simulink model "HRES_ORC_PEM"  (R2025b)
settings: Solver=ode23t  StartTime=0.0  StopTime=35000  MaxStep=1728  RelTol=1e-3
model workspace (MAT data in the model file):
  CND_L = 10
  CND_T0 = 333.15
  CND_d = 0.012
  CND_n = 20
  CND_p0 = 150000
  GAS_Tmax = 430
  GAS_dT = 20
  GAS_kb = 0.04
  GAS_ki = 0.002
  GAS_kp = 0.05
  GAS_min = 0.02
  GAS_total = 5
  GAS_u0 = 0.05
  HRS_L = 10
  HRS_LG = 1
  HRS_d = 0.012
  HRS_n = 6
  HRS_nG = 25
  HRS_p0 = 0.3
  HRS_x0 = 0.2
  NOZ_kb = 0.025
  NOZ_ki = 0.0005
  NOZ_kp = 0.02
  NOZ_min = 0.01
  NOZ_u0 = 0.1
  ORC_T3set = 400
  ORC_Taux = -2
  ORC_Taux0 = 0
  ORC_kb = 0.4
  ORC_ki = 2e-07
  ORC_kp = 5e-07
  ORC_mdot0 = 0.2
  ORC_mmax = 1
  ORC_mmin = 0.01
  ORC_pset_MPa = 1
  RCV_V = 0.2
  RCV_frac0 = 0.5
  RCV_p0 = 0.15
  RCV_tau = 0.1
  TRB_Tref = 400
  TRB_mdot = 0.6
  TRB_pr = 6
values from neighbouring files (symbols this model uses):
  R_h2 = 4.12    [run_simulation.m]
libraries: fl_lib x62, nesl_utility x56, SimscapeFluids_lib x9, slpidlib x4, ee_lib x2
(part 5 of 5)

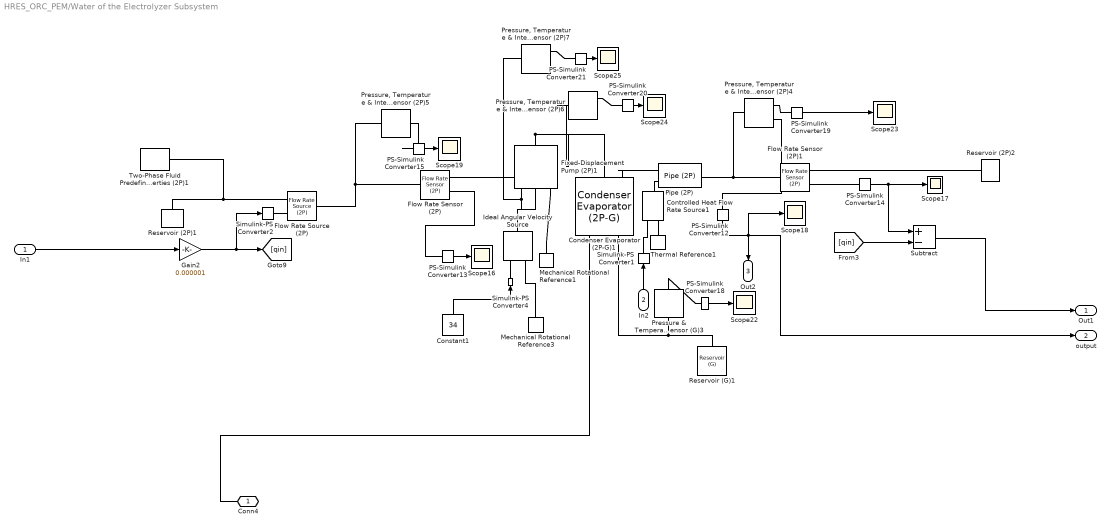
== system HRES_ORC_PEM/Water of the Electrolyzer Subsystem ==
  In1 : Inport
  In2 : Inport  Port=2
  Condenser Evaporator (2P-G)1 : SimscapeFluids_lib/Heat Exchangers/Two-Phase Fluid - Gas/Condenser Evaporator (2P-G)  flow_arrangement=fluids.heat_exchangers.enum.FlowArrangement2PG.Cross  cross_flow_arrangement=fluids.heat_exchangers.enum.CrossFlowArrangement2PG.UnmixedUnmixed  R_wall=0 K/kW  wall_thermal_mass=false  mass_wall=1 kg  cp_wall=490 J/(K*kg)  area_A1=0.01 m^2  area_B1=0.01 m^2  area_A2=0.01 m^2  area_B2=0.01 m^2  tube_num_2P=20  tube_length_2P=1 m  tube_cross_section_2P=fluids.heat_exchangers.enum.TubeCrossSection.Circular  tube_diameter_2P=0.1 m  tube_width_2P=0.05 m  tube_height_2P=0.05 m  tube_inner_diameter_2P=0.05 m  tube_outer_diameter_2P=0.1 m  tube_flow_area_2P=0.002 m^2  tube_wetted_perimeter_2P=0.15 m  tube_heat_perimeter_2P=0.15 m  tube_pressure_loss_spec_2P=fluids.heat_exchangers.enum.TubePressureLossSpec2P.Haaland  tube_loss_coeff_2P=10  tube_local_pressure_loss_spec_2P=fluids.heat_exchangers.enum.LocalLossSpec.AggregateLength  tube_length_add_2P=0.1 m  tube_local_loss_coefficient_2P=0.1  tube_roughness_pressure_2P=15e-6 m  tube_Re_lam_pressure_2P=2000  tube_Re_tur_pressure_2P=4000  tube_shape_factor_generic_2P=64  tube_heat_coeff_spec_2P=fluids.heat_exchangers.enum.TubeHeatCoeffSpec2P.GneilinskiCavalliniZecchin  tube_colburn_coeff_liq_2P=[.023, .8, .33]  tube_colburn_coeff_mix_2P=[.05, .8, .33]  tube_colburn_coeff_vap_2P=[.023, .8, .33]  tube_roughness_heat_2P=15e-6 m  tube_Re_lam_heat_2P=2000  tube_Re_tur_heat_2P=4000  tube_Nu_lam_generic_2P=3.66  fouling_factor_2P=0.1 K*m^2/kW  fin_area_2P=0 m^2  fin_efficiency_2P=0.5  energy_spec_2P=foundation.enum.energy_spec.temperature  p_init_2P=0.6 MPa  T_init_2P=293.15 K  x_init_2P=0.5  alpha_init_2P=0.5  h_init_2P=1500 kJ/kg  u_init_2P=1500 kJ/kg  flow_geometry_G=fluids.heat_exchangers.enum.FlowGeometryG.InsideTubes  tube_num_G=20  tube_length_G=1 m  tube_cross_section_G=fluids.heat_exchangers.enum.TubeCrossSection.Circular  tube_diameter_G=0.05 m  tube_width_G=0.05 m  tube_height_G=0.05 m  tube_inner_diameter_G=0.05 m  tube_outer_diameter_G=0.1 m  tube_flow_area_G=0.002 m^2  tube_wetted_perimeter_G=0.15 m  tube_heat_perimeter_G=0.15 m  tube_pressure_loss_spec_G=fluids.heat_exchangers.enum.TubePressureLossSpec.Haaland  tube_loss_coeff_G=10  tube_local_pressure_loss_spec_G=fluids.heat_exchangers.enum.LocalLossSpec.AggregateLength  tube_length_add_G=0.1 m  tube_local_loss_coefficient_G=0.1  tube_roughness_pressure_G=15e-6 m  tube_Re_lam_pressure_G=2000  tube_Re_tur_pressure_G=4000  tube_shape_factor_generic_G=64  tube_heat_coeff_spec_G=fluids.heat_exchangers.enum.TubeHeatCoeffSpec.Gneilinski  tube_colburn_coeff_G=[.023, .8, .33]  tube_roughness_heat_G=15e-6 m  tube_Re_lam_heat_G=2000  tube_Re_tur_heat_G=4000  tube_Nu_lam_generic_G=3.66  bank_arrangement_G=fluids.heat_exchangers.enum.BankArrangement.Inline  bank_num_rows_G=5  bank_tubes_per_row_G=5  bank_width_G=1 m  bank_tube_diameter_G=0.05 m  bank_longitudinal_pitch_G=0.15 m  bank_transverse_pitch_G=0.15 m  bank_pressure_loss_spec_G=fluids.heat_exchangers.enum.BankPressureLossSpec.Martin  bank_euler_G=10  bank_heat_coeff_spec_G=fluids.heat_exchangers.enum.BankHeatCoeffSpec.Martin  bank_colburn_coeff_G=[.27, .63, .36]  generic_flow_area_G=0.01 m^2  generic_heat_area_G=2 m^2  generic_volume_G=0.05 m^3  generic_loss_coeff_G=10  generic_colburn_coeff_G=[.023, .8, .33]  fouling_factor_G=0.1 K*m^2/kW  fin_area_G=0 m^2  fin_efficiency_G=0.5  p_init_G=0.101325 MPa  T_init_G=250 K
      settings: InternalSimscapePortConfiguration="{\"Bottom\":[],\"Left\":[{\"id\":\"A1\",\"label\":\"A1\",\"type\":\"foundation.two_phase_fluid.two_phase_fluid\"},{\"id\":\"B1\",\"label\":\"B1\",\"type\":\"foundation.two_phase_fluid.two_phase_fluid\"}],\"Right\":[{\"id\":\"A2\",\"label\":\"A2\",\"type\":\"foundation.gas.gas\"},{\"id\":\"B2\",\"label\":\"B2\",\"type\":\"foundation.gas.gas\"}],\"Top\":[{\"id\":\"Z\",\"label\":\"Z\",\"type\":\"output\"}]}"
  Constant1 : Constant  Value=34
  Controlled Heat Flow Rate Source1 : fl_lib/Thermal/Thermal Sources/Controlled Heat Flow Rate Source
  Fixed-Displacement Pump (2P)1 : SimscapeFluids_lib/Two-Phase Fluid/Fluid Machines/Fixed-Displacement Pump (2P)  leakage_friction_spec=fluids.two_phase_fluid.fluid_machines.enum.PumpMotorLossSpec.Analytical  displacement=20 cm^3/rev  omega_nominal=10 rad/s  p_nominal=0.3 MPa  mu_nominal=0.9 cP  vol_eff_nominal=0.85  mech_eff_nominal=0.80  no_load_torque=0 N*m  p_diff_eff_TLU=[.1, 1, 2] MPa  omega_eff_TLU=[250, 500, 1000, 2000, 3000, 4000] rpm  vol_eff_TLU=[.816, .908, .954, .977, .981, .984; .325, .663, .831, .916, .925, .946; .137, .568, .78, .892, .893, .91]  mech_eff_TLU=[.996, .996, .996, .996, .996, .996; .988, .989, .989, .989, .989, .99; .981, .981, .982, .982, .983, .984]  p_diff_loss_TLU=[.1, 1, 2] MPa  omega_loss_TLU=[250, 500, 1000, 2000, 3000, 4000] rpm  vol_loss_TLU=1e-3 * [.023, .023, .023, .023, .0285, .032; .0844, .0842, .0845, .084, .1125, .108; .1079, .108, .11, .108, .1605, .18] m^3/s  mech_loss_TLU=[.002, .002, .002, .002, .002, .002; .0607, .0556, .0556, .0556, .0556, .0505; .1937, .1937, .1833, .1833, .1729, .1626] N*m  vol_eff_min=1e-3  vol_eff_max=1  mech_eff_min=1e-3  mech_eff_max=1  pressure_threshold=1e-3 MPa  omega_threshold=100 rpm  area=0.001 m^2  liquid_check=simscape.enum.assert.action.warn  supplied_range_check=simscape.enum.assert.action.none  pump_mode_check=simscape.enum.assert.action.none
      settings: LogSimulationData=on  InternalSimscapePortConfiguration="{\"Bottom\":[{\"id\":\"A\",\"label\":\"A\",\"type\":\"foundation.two_phase_fluid.two_phase_fluid\"}],\"Left\":[],\"Right\":[{\"id\":\"R\",\"label\":\"R\",\"type\":\"foundation.mechanical.rotational.rotational\"},{\"id\":\"C\",\"label\":\"C\",\"type\":\"foundation.mechanical.rotational.rotational\"}],\"Top\":[{\"id\":\"B\",\"label\":\"B\",\"type\":\"foundation.two_phase_fluid.two_phase_fluid\"}]}"
  Flow Rate Sensor (2P) : fl_lib/Two-Phase Fluid/Sensors/Flow Rate Sensor (2P)  mass_flow_measure=true  volumetric_flow_measure=false  energy_flow_measure=false
      settings: InternalSimscapePortConfiguration="{\"Bottom\":[],\"Left\":[{\"id\":\"A\",\"label\":\"A\",\"type\":\"foundation.two_phase_fluid.two_phase_fluid\"}],\"Right\":[{\"id\":\"B\",\"label\":\"B\",\"type\":\"foundation.two_phase_fluid.two_phase_fluid\"},{\"id\":\"M\",\"label\":\"M\",\"type\":\"output\"}],\"Top\":[]}"
  Flow Rate Sensor (2P)1 : fl_lib/Two-Phase Fluid/Sensors/Flow Rate Sensor (2P)  mass_flow_measure=false  volumetric_flow_measure=true  energy_flow_measure=false
      settings: InternalSimscapePortConfiguration="{\"Bottom\":[],\"Left\":[{\"id\":\"A\",\"label\":\"A\",\"type\":\"foundation.two_phase_fluid.two_phase_fluid\"}],\"Right\":[{\"id\":\"B\",\"label\":\"B\",\"type\":\"foundation.two_phase_fluid.two_phase_fluid\"},{\"id\":\"V\",\"label\":\"V\",\"type\":\"output\"}],\"Top\":[]}"
  Flow Rate Source (2P) : fl_lib/Two-Phase Fluid/Sources/Flow Rate Source (2P)  source_type=foundation.enum.constant_controlled.controlled  flow_type=foundation.enum.mass_volumetric_flow.mass  mass_flow=0 kg/s  volumetric_flow=0 m^3/s  power_spec=foundation.enum.power_spec.isentropic  area_A=0.01 m^2  area_B=0.01 m^2
      settings: InternalSimscapePortConfiguration="{\"Bottom\":[],\"Left\":[{\"id\":\"A\",\"label\":\"A\",\"type\":\"foundation.two_phase_fluid.two_phase_fluid\"},{\"id\":\"M\",\"label\":\"M\",\"type\":\"input\"}],\"Right\":[{\"id\":\"B\",\"label\":\"B\",\"type\":\"foundation.two_phase_fluid.two_phase_fluid\"}],\"Top\":[]}"
  Gain2 : Gain  Gain=0.000001
  Ideal Angular Velocity Source : fl_lib/Mechanical/Mechanical Sources/Ideal Angular Velocity Source
  Mechanical Rotational Reference1 : fl_lib/Mechanical/Rotational Elements/Mechanical Rotational Reference
  Mechanical Rotational Reference3 : fl_lib/Mechanical/Rotational Elements/Mechanical Rotational Reference
  PS-Simulink Converter12 : nesl_utility/PS-Simulink Converter  PhysicalDomain=network_engine_domain  SubClassName=ps_output  LeftPortType=input  RightPortType=output  PseudoPeriodic=off  Frequencies=[]  VectorFormat=inherit  Unit=K  AffineConversion=off
  PS-Simulink Converter13 : nesl_utility/PS-Simulink Converter  PhysicalDomain=network_engine_domain  SubClassName=ps_output  LeftPortType=input  RightPortType=output  PseudoPeriodic=off  Frequencies=[]  VectorFormat=inherit  Unit=inherit  AffineConversion=off
  PS-Simulink Converter14 : nesl_utility/PS-Simulink Converter  PhysicalDomain=network_engine_domain  SubClassName=ps_output  LeftPortType=input  RightPortType=output  PseudoPeriodic=off  Frequencies=[]  VectorFormat=inherit  Unit=m^3/s  AffineConversion=off
  PS-Simulink Converter15 : nesl_utility/PS-Simulink Converter  PhysicalDomain=network_engine_domain  SubClassName=ps_output  LeftPortType=input  RightPortType=output  PseudoPeriodic=off  Frequencies=[]  VectorFormat=inherit  Unit=inherit  AffineConversion=off
  PS-Simulink Converter18 : nesl_utility/PS-Simulink Converter  PhysicalDomain=network_engine_domain  SubClassName=ps_output  LeftPortType=input  RightPortType=output  PseudoPeriodic=off  Frequencies=[]  VectorFormat=inherit  Unit=K  AffineConversion=off
  PS-Simulink Converter19 : nesl_utility/PS-Simulink Converter  PhysicalDomain=network_engine_domain  SubClassName=ps_output  LeftPortType=input  RightPortType=output  PseudoPeriodic=off  Frequencies=[]  VectorFormat=inherit  Unit=inherit  AffineConversion=off
  PS-Simulink Converter20 : nesl_utility/PS-Simulink Converter  PhysicalDomain=network_engine_domain  SubClassName=ps_output  LeftPortType=input  RightPortType=output  PseudoPeriodic=off  Frequencies=[]  VectorFormat=inherit  Unit=Pa  AffineConversion=off
  PS-Simulink Converter21 : nesl_utility/PS-Simulink Converter  PhysicalDomain=network_engine_domain  SubClassName=ps_output  LeftPortType=input  RightPortType=output  PseudoPeriodic=off  Frequencies=[]  VectorFormat=inherit  Unit=Pa  AffineConversion=off
  Pipe (2P) : fl_lib/Two-Phase Fluid/Elements/Pipe (2P)  length=5 m  area=0.01 m^2  Dh=0.1 m  length_add=0.1 m  roughness=15e-6 m  Re_lam=2000  Re_tur=4000  shape_factor=64  Nu_lam=3.66  inertia=false  energy_spec=foundation.enum.energy_spec.temperature  p_init=0.101325 MPa  T_init=293.15 K  x_init=0.5  alpha_init=0.5  h_init=1500 kJ/kg  u_init=1500 kJ/kg  mdot_init=0 kg/s  time_constant=0.1 s
      settings: InternalSimscapePortConfiguration="{\"Bottom\":[],\"Left\":[{\"id\":\"A\",\"label\":\"A\",\"type\":\"foundation.two_phase_fluid.two_phase_fluid\"},{\"id\":\"H\",\"label\":\"H\",\"type\":\"foundation.thermal.thermal\"}],\"Right\":[{\"id\":\"B\",\"label\":\"B\",\"type\":\"foundation.two_phase_fluid.two_phase_fluid\"}],\"Top\":[]}"
  Pressure & Temperature Sensor (G)3 : fl_lib/Gas/Sensors/Pressure & Temperature Sensor (G)  reference=foundation.enum.MeasurementReference.absolute  pressure=false  pressure_spec=foundation.enum.PressureMeasementSpec.Absolute  temperature=true
      settings: InternalSimscapePortConfiguration="{\"Bottom\":[{\"id\":\"T\",\"label\":\"T\",\"type\":\"output\"}],\"Left\":[{\"id\":\"A\",\"label\":\"A\",\"type\":\"foundation.gas.gas\"}],\"Right\":[],\"Top\":[]}"
  "Pressure, Temperature & Internal Energy Sensor (2P)4" : fl_lib/Two-Phase Fluid/Sensors/Pressure, Temperature & Internal Energy Sensor (2P)  reference=foundation.enum.MeasurementReference.absolute  pressure=true  pressure_spec=foundation.enum.PressureMeasementSpec.Absolute  temperature=true  internal_energy=false
      settings: InternalSimscapePortConfiguration="{\"Bottom\":[{\"id\":\"T\",\"label\":\"T\",\"type\":\"output\"}],\"Left\":[{\"id\":\"A\",\"label\":\"A\",\"type\":\"foundation.two_phase_fluid.two_phase_fluid\"}],\"Right\":[{\"id\":\"Pa\",\"label\":\"Pa\",\"type\":\"output\"}],\"Top\":[]}"
  "Pressure, Temperature & Internal Energy Sensor (2P)5" : fl_lib/Two-Phase Fluid/Sensors/Pressure, Temperature & Internal Energy Sensor (2P)  reference=foundation.enum.MeasurementReference.absolute  pressure=false  pressure_spec=foundation.enum.PressureMeasementSpec.Absolute  temperature=true  internal_energy=false
      settings: InternalSimscapePortConfiguration="{\"Bottom\":[{\"id\":\"T\",\"label\":\"T\",\"type\":\"output\"}],\"Left\":[{\"id\":\"A\",\"label\":\"A\",\"type\":\"foundation.two_phase_fluid.two_phase_fluid\"}],\"Right\":[],\"Top\":[]}"
  "Pressure, Temperature & Internal Energy Sensor (2P)6" : fl_lib/Two-Phase Fluid/Sensors/Pressure, Temperature & Internal Energy Sensor (2P)  reference=foundation.enum.MeasurementReference.absolute  pressure=true  pressure_spec=foundation.enum.PressureMeasementSpec.Absolute  temperature=true  internal_energy=false
      settings: InternalSimscapePortConfiguration="{\"Bottom\":[{\"id\":\"T\",\"label\":\"T\",\"type\":\"output\"}],\"Left\":[{\"id\":\"A\",\"label\":\"A\",\"type\":\"foundation.two_phase_fluid.two_phase_fluid\"}],\"Right\":[{\"id\":\"Pa\",\"label\":\"Pa\",\"type\":\"output\"}],\"Top\":[]}"
  "Pressure, Temperature & Internal Energy Sensor (2P)7" : fl_lib/Two-Phase Fluid/Sensors/Pressure, Temperature & Internal Energy Sensor (2P)  reference=foundation.enum.MeasurementReference.absolute  pressure=true  pressure_spec=foundation.enum.PressureMeasementSpec.Absolute  temperature=true  internal_energy=false
      settings: InternalSimscapePortConfiguration="{\"Bottom\":[{\"id\":\"T\",\"label\":\"T\",\"type\":\"output\"}],\"Left\":[{\"id\":\"A\",\"label\":\"A\",\"type\":\"foundation.two_phase_fluid.two_phase_fluid\"}],\"Right\":[{\"id\":\"Pa\",\"label\":\"Pa\",\"type\":\"output\"}],\"Top\":[]}"
  Reservoir (2P)1 : fl_lib/Two-Phase Fluid/Elements/Reservoir (2P)  pressure_spec=foundation.enum.ReservoirPressureSpec2P.Specified  reservoir_pressure=1 bar  reservoir_condensing_temperature=373.15 K  reservoir_evaporating_temperature=373.15 K  energy_spec=foundation.enum.ReservoirEnergySpec2P.Temperature  reservoir_temperature=300 K  reservoir_quality=0.5  reservoir_void_fraction=0.5  reservoir_enthalpy=1500 kJ/kg  reservoir_internal_energy=1500 kJ/kg  reservoir_subcooling=5 deltaK  reservoir_superheating=5 deltaK  area_A=0.01 m^2
  Reservoir (2P)2 : fl_lib/Two-Phase Fluid/Elements/Reservoir (2P)  pressure_spec=foundation.enum.ReservoirPressureSpec2P.Specified  reservoir_pressure=5 bar  reservoir_condensing_temperature=373.15 K  reservoir_evaporating_temperature=373.15 K  energy_spec=foundation.enum.ReservoirEnergySpec2P.Temperature  reservoir_temperature=370 K  reservoir_quality=0.5  reservoir_void_fraction=0.5  reservoir_enthalpy=1500 kJ/kg  reservoir_internal_energy=1500 kJ/kg  reservoir_subcooling=5 deltaK  reservoir_superheating=5 deltaK  area_A=0.01 m^2
  Reservoir (G)1 : fl_lib/Gas/Elements/Reservoir (G)  pressure_spec=foundation.enum.pressure_spec.atmospheric  reservoir_pressure=0.101325 MPa  reservoir_temperature=293.15 K  area_A=0.01 m^2
  Scope{16..19,22..25} (8 alike) : Scope
      Scope16 settings: ActiveDisplayYMinimum=-4.6224964079817441E-7  ActiveDisplayYMaximum=4.160246767183571E-6  DataLoggingVariableName=ScopeData18
      Scope17 settings: ActiveDisplayYMinimum=-0.00043435582595641739  ActiveDisplayYMaximum=0.0035069615419707017  DataLoggingVariableName=ScopeData19
      Scope18 settings: ActiveDisplayYMinimum=296.23361130845234  ActiveDisplayYMaximum=380.90999792555522  DataLoggingVariableName=ScopeData15
      Scope19 settings: ActiveDisplayYMinimum=269.69619495924803  ActiveDisplayYMaximum=487.04134680243965  DataLoggingVariableName=ScopeData17
      Scope22 settings: ActiveDisplayYMinimum=-544.89033893414171  ActiveDisplayYMaximum=1096.9615501303642  DataLoggingVariableName=ScopeData22
      Scope23 settings: ActiveDisplayYMinimum=0.099971820776618758  ActiveDisplayYMaximum=0.10001711054963275  DataLoggingVariableName=ScopeData23
      Scope24 settings: ActiveDisplayYMinimum=499999.999811996  ActiveDisplayYMaximum=500000.00715155876  DataLoggingVariableName=ScopeData24
      Scope25 settings: ActiveDisplayYMinimum=499999.999811996  ActiveDisplayYMaximum=500000.00715155876  DataLoggingVariableName=ScopeData25
  Simulink-PS Converter1 : nesl_utility/Simulink-PS Converter  PhysicalDomain=network_engine_domain  SubClassName=ps_input  LeftPortType=input  RightPortType=output  PseudoPeriodic=off  Frequencies=[]  NoiseDistribution=none  NoiseParameters=[]  Unit=W  AffineConversion=off  FilteringAndDerivatives=provide  SimscapeFilterOrder=1  InputFilterTimeConstant=0.001  UdotUserProvided=0
  Simulink-PS Converter2 : nesl_utility/Simulink-PS Converter  PhysicalDomain=network_engine_domain  SubClassName=ps_input  LeftPortType=input  RightPortType=output  PseudoPeriodic=off  Frequencies=[]  NoiseDistribution=none  NoiseParameters=[]  Unit=1  AffineConversion=off  FilteringAndDerivatives=provide  SimscapeFilterOrder=1  InputFilterTimeConstant=0.001  UdotUserProvided=0
  Simulink-PS Converter4 : nesl_utility/Simulink-PS Converter  PhysicalDomain=network_engine_domain  SubClassName=ps_input  LeftPortType=input  RightPortType=output  PseudoPeriodic=off  Frequencies=[]  NoiseDistribution=none  NoiseParameters=[]  Unit=1  AffineConversion=off  FilteringAndDerivatives=provide  SimscapeFilterOrder=1  InputFilterTimeConstant=0.001  UdotUserProvided=0
  Subtract : Sum  Inputs=+-
  Thermal Reference1 : fl_lib/Thermal/Thermal Elements/Thermal Reference
  Two-Phase Fluid Predefined Properties (2P)1 : SimscapeFluids_lib/Two-Phase Fluid/Utilities/Two-Phase Fluid Predefined Properties (2P)  fluid=fluids.two_phase_fluid.utilities.enum.Fluid.Water  p_atm=0.101325 MPa  properties_range_check=simscape.enum.assert.action.error  q_rev=0.01 Pa
  Conn4 : PMIOPort  Side=Right
  Out1 : Outport
  output : Outport  Port=2
  Out2 : Outport  Port=3
  wires:
  PS-Simulink Converter13/1 -> Scope16/1
  PS-Simulink Converter15/1 -> Scope19/1
  PS-Simulink Converter21/1 -> Scope25/1
  PS-Simulink Converter19/1 -> Scope23/1
  PS-Simulink Converter12/1 -> output/1, Scope18/1, Out2/1
  PS-Simulink Converter20/1 -> Scope24/1
  Constant1/1 -> Simulink-PS Converter4/1
  PS-Simulink Converter14/1 -> Subtract/1, Scope17/1
  PS-Simulink Converter18/1 -> Scope22/1
  [qin] -> Subtract/2
  In1/1 -> Gain2/1
  Gain2/1 -> Simulink-PS Converter2/1, [qin]
  Subtract/1 -> Out1/1
  In2/1 -> Simulink-PS Converter1/1
  connections:
  PS-Simulink Converter12/LConn1 -- "Pressure, Temperature & Internal Energy Sensor (2P)4"/RConn2
  "Pressure, Temperature & Internal Energy Sensor (2P)5"/LConn1 -- Flow Rate Sensor (2P)/LConn1 -- Flow Rate Source (2P)/RConn1
  Reservoir (G)1/LConn1 -- Pressure & Temperature Sensor (G)3/LConn1 -- Condenser Evaporator (2P-G)1/RConn1
  Mechanical Rotational Reference3/LConn1 -- Ideal Angular Velocity Source/RConn2
  Ideal Angular Velocity Source/RConn1 -- Simulink-PS Converter4/RConn1
  Two-Phase Fluid Predefined Properties (2P)1/RConn1 -- Reservoir (2P)1/LConn1 -- Flow Rate Source (2P)/LConn1
  PS-Simulink Converter21/LConn1 -- "Pressure, Temperature & Internal Energy Sensor (2P)7"/RConn1
  Mechanical Rotational Reference1/LConn1 -- Fixed-Displacement Pump (2P)1/RConn1
  PS-Simulink Converter20/LConn1 -- "Pressure, Temperature & Internal Energy Sensor (2P)6"/RConn1
  Flow Rate Sensor (2P)/RConn2 -- PS-Simulink Converter13/LConn1
  PS-Simulink Converter15/LConn1 -- "Pressure, Temperature & Internal Energy Sensor (2P)5"/RConn1
  Flow Rate Source (2P)/LConn2 -- Simulink-PS Converter2/RConn1
  PS-Simulink Converter19/LConn1 -- "Pressure, Temperature & Internal Energy Sensor (2P)4"/RConn1
  "Pressure, Temperature & Internal Energy Sensor (2P)4"/LConn1 -- Flow Rate Sensor (2P)1/LConn1 -- Pipe (2P)/RConn1
  Pipe (2P)/LConn1 -- Condenser Evaporator (2P-G)1/LConn1
  Pressure & Temperature Sensor (G)3/RConn1 -- PS-Simulink Converter18/LConn1
  Fixed-Displacement Pump (2P)1/RConn3 -- Flow Rate Sensor (2P)/RConn1 -- "Pressure, Temperature & Internal Energy Sensor (2P)7"/LConn1
  PS-Simulink Converter14/LConn1 -- Flow Rate Sensor (2P)1/RConn2
  Fixed-Displacement Pump (2P)1/LConn1 -- "Pressure, Temperature & Internal Energy Sensor (2P)6"/LConn1 -- Condenser Evaporator (2P-G)1/LConn2
  Conn4/RConn1 -- Condenser Evaporator (2P-G)1/RConn2
  Flow Rate Sensor (2P)1/RConn1 -- Reservoir (2P)2/LConn1
  Fixed-Displacement Pump (2P)1/RConn2 -- Ideal Angular Velocity Source/LConn1
  Thermal Reference1/LConn1 -- Controlled Heat Flow Rate Source1/RConn2
  Simulink-PS Converter1/RConn1 -- Controlled Heat Flow Rate Source1/RConn1
  Controlled Heat Flow Rate Source1/LConn1 -- Pipe (2P)/LConn2

== system HRES_ORC_PEM/ORC/Load Torque ==
  In1 : Inport
  In2 : Inport  Port=2
  In3 : Inport  Port=3
  Switch : Switch  Threshold=1000  SaturateOnIntegerOverflow=off  InputSameDT=off
  Out1 : Outport
  wires:
  In1/1 -> Switch/3
  Switch/1 -> Out1/1
  In2/1 -> Switch/2
  In3/1 -> Switch/1

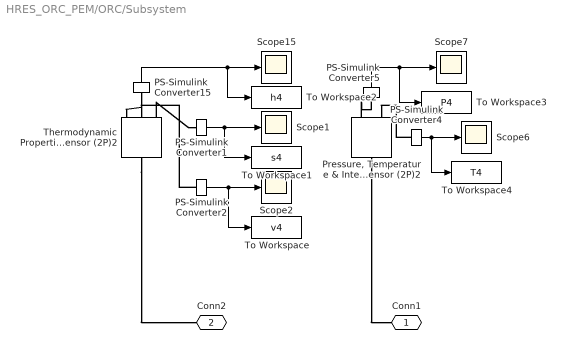
== system HRES_ORC_PEM/ORC/Subsystem ==
  PS-Simulink Converter1 : nesl_utility/PS-Simulink Converter  PhysicalDomain=network_engine_domain  SubClassName=ps_output  LeftPortType=input  RightPortType=output  PseudoPeriodic=off  Frequencies=[]  VectorFormat=inherit  Unit=J/(kg*K)  AffineConversion=off
  PS-Simulink Converter15 : nesl_utility/PS-Simulink Converter  PhysicalDomain=network_engine_domain  SubClassName=ps_output  LeftPortType=input  RightPortType=output  PseudoPeriodic=off  Frequencies=[]  VectorFormat=inherit  Unit=kJ/kg  AffineConversion=off
  PS-Simulink Converter2 : nesl_utility/PS-Simulink Converter  PhysicalDomain=network_engine_domain  SubClassName=ps_output  LeftPortType=input  RightPortType=output  PseudoPeriodic=off  Frequencies=[]  VectorFormat=inherit  Unit=m^3/kg  AffineConversion=off
  PS-Simulink Converter4 : nesl_utility/PS-Simulink Converter  PhysicalDomain=network_engine_domain  SubClassName=ps_output  LeftPortType=input  RightPortType=output  PseudoPeriodic=off  Frequencies=[]  VectorFormat=inherit  Unit=K  AffineConversion=off
  PS-Simulink Converter5 : nesl_utility/PS-Simulink Converter  PhysicalDomain=network_engine_domain  SubClassName=ps_output  LeftPortType=input  RightPortType=output  PseudoPeriodic=off  Frequencies=[]  VectorFormat=inherit  Unit=Pa  AffineConversion=off
  "Pressure, Temperature & Internal Energy Sensor (2P)2" : fl_lib/Two-Phase Fluid/Sensors/Pressure, Temperature & Internal Energy Sensor (2P)  reference=foundation.enum.MeasurementReference.absolute  pressure=true  pressure_spec=foundation.enum.PressureMeasementSpec.Absolute  temperature=true  internal_energy=false
      settings: InternalSimscapePortConfiguration="{\"Bottom\":[{\"id\":\"T\",\"label\":\"T\",\"type\":\"output\"}],\"Left\":[{\"id\":\"A\",\"label\":\"A\",\"type\":\"foundation.two_phase_fluid.two_phase_fluid\"}],\"Right\":[{\"id\":\"Pa\",\"label\":\"Pa\",\"type\":\"output\"}],\"Top\":[]}"
  Scope{1..2,6..7,15} (5 alike) : Scope
      Scope1 settings: ActiveDisplayYMinimum=375.93552600794726  ActiveDisplayYMaximum=401.12975249571122  DataLoggingVariableName=ScopeData27
      Scope15 settings: ActiveDisplayYMinimum=260.896690836373  ActiveDisplayYMaximum=388.3546236466708  DataLoggingVariableName=ScopeData20
      Scope2 settings: ActiveDisplayYMinimum=375.93552600794726  ActiveDisplayYMaximum=401.12975249571122  DataLoggingVariableName=ScopeData28
      Scope6 settings: ActiveDisplayYMinimum=-1  ActiveDisplayYMaximum=1  DataLoggingVariableName=ScopeData6
      Scope7 settings: ActiveDisplayYMinimum=287076.80367816926  ActiveDisplayYMaximum=1.2873113409355804E+6  DataLoggingVariableName=ScopeData7
  Thermodynamic Properties Sensor (2P)2 : fl_lib/Two-Phase Fluid/Sensors/Thermodynamic Properties Sensor (2P)  temperature=false  enthalpy=true  density=false  specific_volume=true  entropy=true
      settings: InternalSimscapePortConfiguration="{\"Bottom\":[{\"id\":\"V\",\"label\":\"v\",\"type\":\"output\"},{\"id\":\"S\",\"label\":\"s\",\"type\":\"output\"}],\"Left\":[{\"id\":\"A\",\"label\":\"A\",\"type\":\"foundation.two_phase_fluid.two_phase_fluid\"}],\"Right\":[{\"id\":\"H\",\"label\":\"h\",\"type\":\"output\"}],\"Top\":[]}"
  To Workspace : ToWorkspace  VariableName=v4  SampleTime=-1
  To Workspace1 : ToWorkspace  VariableName=s4  SampleTime=-1
  To Workspace2 : ToWorkspace  VariableName=h4  SampleTime=-1
  To Workspace3 : ToWorkspace  VariableName=P4  SampleTime=-1
  To Workspace4 : ToWorkspace  VariableName=T4  SampleTime=-1
  Conn1 : PMIOPort  Side=Left
  Conn2 : PMIOPort  Port=2  Side=Left
  wires:
  PS-Simulink Converter15/1 -> To Workspace2/1, Scope15/1
  PS-Simulink Converter5/1 -> To Workspace3/1, Scope7/1
  PS-Simulink Converter1/1 -> To Workspace1/1, Scope1/1
  PS-Simulink Converter2/1 -> To Workspace/1, Scope2/1
  PS-Simulink Converter4/1 -> To Workspace4/1, Scope6/1
  connections:
  PS-Simulink Converter4/LConn1 -- "Pressure, Temperature & Internal Energy Sensor (2P)2"/RConn2
  PS-Simulink Converter15/LConn1 -- Thermodynamic Properties Sensor (2P)2/RConn1
  Thermodynamic Properties Sensor (2P)2/LConn1 -- Conn2/RConn1
  "Pressure, Temperature & Internal Energy Sensor (2P)2"/RConn1 -- PS-Simulink Converter5/LConn1
  "Pressure, Temperature & Internal Energy Sensor (2P)2"/LConn1 -- Conn1/RConn1
  Thermodynamic Properties Sensor (2P)2/RConn3 -- PS-Simulink Converter1/LConn1
  PS-Simulink Converter2/LConn1 -- Thermodynamic Properties Sensor (2P)2/RConn2

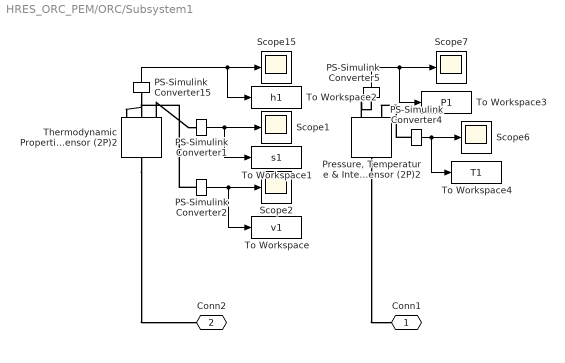
== system HRES_ORC_PEM/ORC/Subsystem1 ==
  PS-Simulink Converter1 : nesl_utility/PS-Simulink Converter  PhysicalDomain=network_engine_domain  SubClassName=ps_output  LeftPortType=input  RightPortType=output  PseudoPeriodic=off  Frequencies=[]  VectorFormat=inherit  Unit=J/(kg*K)  AffineConversion=off
  PS-Simulink Converter15 : nesl_utility/PS-Simulink Converter  PhysicalDomain=network_engine_domain  SubClassName=ps_output  LeftPortType=input  RightPortType=output  PseudoPeriodic=off  Frequencies=[]  VectorFormat=inherit  Unit=kJ/kg  AffineConversion=off
  PS-Simulink Converter2 : nesl_utility/PS-Simulink Converter  PhysicalDomain=network_engine_domain  SubClassName=ps_output  LeftPortType=input  RightPortType=output  PseudoPeriodic=off  Frequencies=[]  VectorFormat=inherit  Unit=m^3/kg  AffineConversion=off
  PS-Simulink Converter4 : nesl_utility/PS-Simulink Converter  PhysicalDomain=network_engine_domain  SubClassName=ps_output  LeftPortType=input  RightPortType=output  PseudoPeriodic=off  Frequencies=[]  VectorFormat=inherit  Unit=K  AffineConversion=off
  PS-Simulink Converter5 : nesl_utility/PS-Simulink Converter  PhysicalDomain=network_engine_domain  SubClassName=ps_output  LeftPortType=input  RightPortType=output  PseudoPeriodic=off  Frequencies=[]  VectorFormat=inherit  Unit=Pa  AffineConversion=off
  "Pressure, Temperature & Internal Energy Sensor (2P)2" : fl_lib/Two-Phase Fluid/Sensors/Pressure, Temperature & Internal Energy Sensor (2P)  reference=foundation.enum.MeasurementReference.absolute  pressure=true  pressure_spec=foundation.enum.PressureMeasementSpec.Absolute  temperature=true  internal_energy=false
      settings: InternalSimscapePortConfiguration="{\"Bottom\":[{\"id\":\"T\",\"label\":\"T\",\"type\":\"output\"}],\"Left\":[{\"id\":\"A\",\"label\":\"A\",\"type\":\"foundation.two_phase_fluid.two_phase_fluid\"}],\"Right\":[{\"id\":\"Pa\",\"label\":\"Pa\",\"type\":\"output\"}],\"Top\":[]}"
  Scope{1..2,6..7,15} (5 alike) : Scope
      Scope1 settings: ActiveDisplayYMinimum=375.93552600794726  ActiveDisplayYMaximum=401.12975249571122  DataLoggingVariableName=ScopeData27
      Scope15 settings: ActiveDisplayYMinimum=375.93552600794726  ActiveDisplayYMaximum=401.12975249571122  DataLoggingVariableName=ScopeData20
      Scope2 settings: ActiveDisplayYMinimum=375.93552600794726  ActiveDisplayYMaximum=401.12975249571122  DataLoggingVariableName=ScopeData28
      Scope6 settings: ActiveDisplayYMinimum=326.971835800604  ActiveDisplayYMaximum=385.06077237390258  DataLoggingVariableName=ScopeData6
      Scope7 settings: ActiveDisplayYMinimum=287076.80367816926  ActiveDisplayYMaximum=1.2873113409355804E+6  DataLoggingVariableName=ScopeData7
  Thermodynamic Properties Sensor (2P)2 : fl_lib/Two-Phase Fluid/Sensors/Thermodynamic Properties Sensor (2P)  temperature=false  enthalpy=true  density=false  specific_volume=true  entropy=true
      settings: InternalSimscapePortConfiguration="{\"Bottom\":[{\"id\":\"V\",\"label\":\"v\",\"type\":\"output\"},{\"id\":\"S\",\"label\":\"s\",\"type\":\"output\"}],\"Left\":[{\"id\":\"A\",\"label\":\"A\",\"type\":\"foundation.two_phase_fluid.two_phase_fluid\"}],\"Right\":[{\"id\":\"H\",\"label\":\"h\",\"type\":\"output\"}],\"Top\":[]}"
  To Workspace : ToWorkspace  VariableName=v1  SampleTime=-1
  To Workspace1 : ToWorkspace  VariableName=s1  SampleTime=-1
  To Workspace2 : ToWorkspace  VariableName=h1  SampleTime=-1
  To Workspace3 : ToWorkspace  VariableName=P1  SampleTime=-1
  To Workspace4 : ToWorkspace  VariableName=T1  SampleTime=-1
  Conn1 : PMIOPort  Side=Left
  Conn2 : PMIOPort  Port=2  Side=Left
  wires:
  PS-Simulink Converter15/1 -> To Workspace2/1, Scope15/1
  PS-Simulink Converter5/1 -> To Workspace3/1, Scope7/1
  PS-Simulink Converter1/1 -> To Workspace1/1, Scope1/1
  PS-Simulink Converter2/1 -> To Workspace/1, Scope2/1
  PS-Simulink Converter4/1 -> To Workspace4/1, Scope6/1
  connections:
  PS-Simulink Converter4/LConn1 -- "Pressure, Temperature & Internal Energy Sensor (2P)2"/RConn2
  PS-Simulink Converter15/LConn1 -- Thermodynamic Properties Sensor (2P)2/RConn1
  Thermodynamic Properties Sensor (2P)2/LConn1 -- Conn2/RConn1
  "Pressure, Temperature & Internal Energy Sensor (2P)2"/RConn1 -- PS-Simulink Converter5/LConn1
  "Pressure, Temperature & Internal Energy Sensor (2P)2"/LConn1 -- Conn1/RConn1
  Thermodynamic Properties Sensor (2P)2/RConn3 -- PS-Simulink Converter1/LConn1
  PS-Simulink Converter2/LConn1 -- Thermodynamic Properties Sensor (2P)2/RConn2

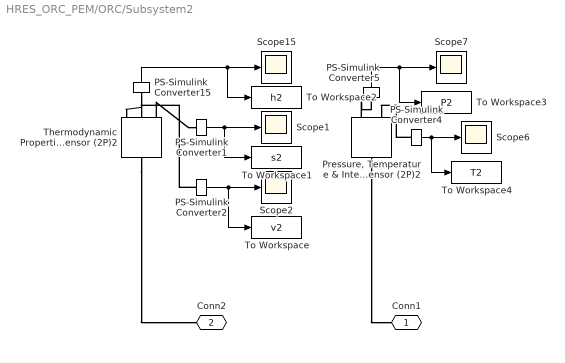
== system HRES_ORC_PEM/ORC/Subsystem2 ==
  PS-Simulink Converter1 : nesl_utility/PS-Simulink Converter  PhysicalDomain=network_engine_domain  SubClassName=ps_output  LeftPortType=input  RightPortType=output  PseudoPeriodic=off  Frequencies=[]  VectorFormat=inherit  Unit=J/(kg*K)  AffineConversion=off
  PS-Simulink Converter15 : nesl_utility/PS-Simulink Converter  PhysicalDomain=network_engine_domain  SubClassName=ps_output  LeftPortType=input  RightPortType=output  PseudoPeriodic=off  Frequencies=[]  VectorFormat=inherit  Unit=kJ/kg  AffineConversion=off
  PS-Simulink Converter2 : nesl_utility/PS-Simulink Converter  PhysicalDomain=network_engine_domain  SubClassName=ps_output  LeftPortType=input  RightPortType=output  PseudoPeriodic=off  Frequencies=[]  VectorFormat=inherit  Unit=m^3/kg  AffineConversion=off
  PS-Simulink Converter4 : nesl_utility/PS-Simulink Converter  PhysicalDomain=network_engine_domain  SubClassName=ps_output  LeftPortType=input  RightPortType=output  PseudoPeriodic=off  Frequencies=[]  VectorFormat=inherit  Unit=K  AffineConversion=off
  PS-Simulink Converter5 : nesl_utility/PS-Simulink Converter  PhysicalDomain=network_engine_domain  SubClassName=ps_output  LeftPortType=input  RightPortType=output  PseudoPeriodic=off  Frequencies=[]  VectorFormat=inherit  Unit=Pa  AffineConversion=off
  "Pressure, Temperature & Internal Energy Sensor (2P)2" : fl_lib/Two-Phase Fluid/Sensors/Pressure, Temperature & Internal Energy Sensor (2P)  reference=foundation.enum.MeasurementReference.absolute  pressure=true  pressure_spec=foundation.enum.PressureMeasementSpec.Absolute  temperature=true  internal_energy=false
      settings: InternalSimscapePortConfiguration="{\"Bottom\":[{\"id\":\"T\",\"label\":\"T\",\"type\":\"output\"}],\"Left\":[{\"id\":\"A\",\"label\":\"A\",\"type\":\"foundation.two_phase_fluid.two_phase_fluid\"}],\"Right\":[{\"id\":\"Pa\",\"label\":\"Pa\",\"type\":\"output\"}],\"Top\":[]}"
  Scope{1..2,6..7,15} (5 alike) : Scope
      Scope1 settings: ActiveDisplayYMinimum=375.93552600794726  ActiveDisplayYMaximum=401.12975249571122  DataLoggingVariableName=ScopeData27
      Scope15 settings: ActiveDisplayYMinimum=259.15754614794685  ActiveDisplayYMaximum=367.56698491549525  DataLoggingVariableName=ScopeData20
      Scope2 settings: ActiveDisplayYMinimum=375.93552600794726  ActiveDisplayYMaximum=401.12975249571122  DataLoggingVariableName=ScopeData28
      Scope6 settings: ActiveDisplayYMinimum=326.971835800604  ActiveDisplayYMaximum=385.06077237390258  DataLoggingVariableName=ScopeData6
      Scope7 settings: ActiveDisplayYMinimum=-546655.63192406553  ActiveDisplayYMaximum=5.9334330333723836E+6  DataLoggingVariableName=ScopeData7
  Thermodynamic Properties Sensor (2P)2 : fl_lib/Two-Phase Fluid/Sensors/Thermodynamic Properties Sensor (2P)  temperature=false  enthalpy=true  density=false  specific_volume=true  entropy=true
      settings: InternalSimscapePortConfiguration="{\"Bottom\":[{\"id\":\"V\",\"label\":\"v\",\"type\":\"output\"},{\"id\":\"S\",\"label\":\"s\",\"type\":\"output\"}],\"Left\":[{\"id\":\"A\",\"label\":\"A\",\"type\":\"foundation.two_phase_fluid.two_phase_fluid\"}],\"Right\":[{\"id\":\"H\",\"label\":\"h\",\"type\":\"output\"}],\"Top\":[]}"
  To Workspace : ToWorkspace  VariableName=v2  SampleTime=-1
  To Workspace1 : ToWorkspace  VariableName=s2  SampleTime=-1
  To Workspace2 : ToWorkspace  VariableName=h2  SampleTime=-1
  To Workspace3 : ToWorkspace  VariableName=P2  SampleTime=-1
  To Workspace4 : ToWorkspace  VariableName=T2  SampleTime=-1
  Conn1 : PMIOPort  Side=Left
  Conn2 : PMIOPort  Port=2  Side=Left
  wires:
  PS-Simulink Converter15/1 -> To Workspace2/1, Scope15/1
  PS-Simulink Converter5/1 -> To Workspace3/1, Scope7/1
  PS-Simulink Converter1/1 -> To Workspace1/1, Scope1/1
  PS-Simulink Converter2/1 -> To Workspace/1, Scope2/1
  PS-Simulink Converter4/1 -> To Workspace4/1, Scope6/1
  connections:
  PS-Simulink Converter4/LConn1 -- "Pressure, Temperature & Internal Energy Sensor (2P)2"/RConn2
  PS-Simulink Converter15/LConn1 -- Thermodynamic Properties Sensor (2P)2/RConn1
  Thermodynamic Properties Sensor (2P)2/LConn1 -- Conn2/RConn1
  "Pressure, Temperature & Internal Energy Sensor (2P)2"/RConn1 -- PS-Simulink Converter5/LConn1
  "Pressure, Temperature & Internal Energy Sensor (2P)2"/LConn1 -- Conn1/RConn1
  Thermodynamic Properties Sensor (2P)2/RConn3 -- PS-Simulink Converter1/LConn1
  PS-Simulink Converter2/LConn1 -- Thermodynamic Properties Sensor (2P)2/RConn2

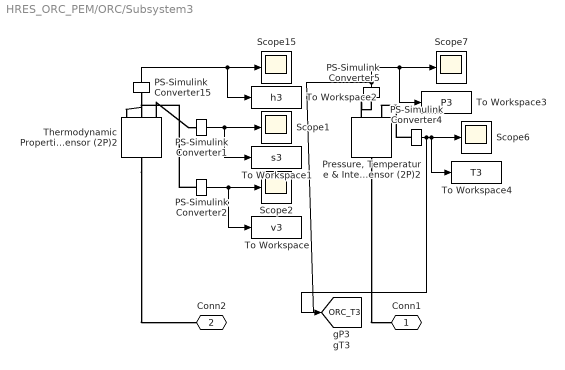
== system HRES_ORC_PEM/ORC/Subsystem3 ==
  PS-Simulink Converter1 : nesl_utility/PS-Simulink Converter  PhysicalDomain=network_engine_domain  SubClassName=ps_output  LeftPortType=input  RightPortType=output  PseudoPeriodic=off  Frequencies=[]  VectorFormat=inherit  Unit=J/(kg*K)  AffineConversion=off
  PS-Simulink Converter15 : nesl_utility/PS-Simulink Converter  PhysicalDomain=network_engine_domain  SubClassName=ps_output  LeftPortType=input  RightPortType=output  PseudoPeriodic=off  Frequencies=[]  VectorFormat=inherit  Unit=kJ/kg  AffineConversion=off
  PS-Simulink Converter2 : nesl_utility/PS-Simulink Converter  PhysicalDomain=network_engine_domain  SubClassName=ps_output  LeftPortType=input  RightPortType=output  PseudoPeriodic=off  Frequencies=[]  VectorFormat=inherit  Unit=m^3/kg  AffineConversion=off
  PS-Simulink Converter4 : nesl_utility/PS-Simulink Converter  PhysicalDomain=network_engine_domain  SubClassName=ps_output  LeftPortType=input  RightPortType=output  PseudoPeriodic=off  Frequencies=[]  VectorFormat=inherit  Unit=K  AffineConversion=off
  PS-Simulink Converter5 : nesl_utility/PS-Simulink Converter  PhysicalDomain=network_engine_domain  SubClassName=ps_output  LeftPortType=input  RightPortType=output  PseudoPeriodic=off  Frequencies=[]  VectorFormat=inherit  Unit=Pa  AffineConversion=off
  "Pressure, Temperature & Internal Energy Sensor (2P)2" : fl_lib/Two-Phase Fluid/Sensors/Pressure, Temperature & Internal Energy Sensor (2P)  reference=foundation.enum.MeasurementReference.absolute  pressure=true  pressure_spec=foundation.enum.PressureMeasementSpec.Absolute  temperature=true  internal_energy=false
      settings: InternalSimscapePortConfiguration="{\"Bottom\":[{\"id\":\"T\",\"label\":\"T\",\"type\":\"output\"}],\"Left\":[{\"id\":\"A\",\"label\":\"A\",\"type\":\"foundation.two_phase_fluid.two_phase_fluid\"}],\"Right\":[{\"id\":\"Pa\",\"label\":\"Pa\",\"type\":\"output\"}],\"Top\":[]}"
  Scope{1..2,6..7,15} (5 alike) : Scope
      Scope1 settings: ActiveDisplayYMinimum=375.93552600794726  ActiveDisplayYMaximum=401.12975249571122  DataLoggingVariableName=ScopeData27
      Scope15 settings: ActiveDisplayYMinimum=257.59523136857871  ActiveDisplayYMaximum=390.72406847398537  DataLoggingVariableName=ScopeData20
      Scope2 settings: ActiveDisplayYMinimum=375.93552600794726  ActiveDisplayYMaximum=401.12975249571122  DataLoggingVariableName=ScopeData28
      Scope6 settings: ActiveDisplayYMinimum=326.971835800604  ActiveDisplayYMaximum=385.06077237390258  DataLoggingVariableName=ScopeData6
      Scope7 settings: ActiveDisplayYMinimum=-546596.57482508838  ActiveDisplayYMaximum=5.9333855039389776E+6  DataLoggingVariableName=ScopeData7
  Thermodynamic Properties Sensor (2P)2 : fl_lib/Two-Phase Fluid/Sensors/Thermodynamic Properties Sensor (2P)  temperature=false  enthalpy=true  density=false  specific_volume=true  entropy=true
      settings: InternalSimscapePortConfiguration="{\"Bottom\":[{\"id\":\"V\",\"label\":\"v\",\"type\":\"output\"},{\"id\":\"S\",\"label\":\"s\",\"type\":\"output\"}],\"Left\":[{\"id\":\"A\",\"label\":\"A\",\"type\":\"foundation.two_phase_fluid.two_phase_fluid\"}],\"Right\":[{\"id\":\"H\",\"label\":\"h\",\"type\":\"output\"}],\"Top\":[]}"
  To Workspace : ToWorkspace  VariableName=v3  SampleTime=-1
  To Workspace1 : ToWorkspace  VariableName=s3  SampleTime=-1
  To Workspace2 : ToWorkspace  VariableName=h3  SampleTime=-1
  To Workspace3 : ToWorkspace  VariableName=P3  SampleTime=-1
  To Workspace4 : ToWorkspace  VariableName=T3  SampleTime=-1
  Conn1 : PMIOPort  Side=Left
  Conn2 : PMIOPort  Port=2  Side=Left
  tag scope: ORC_P3=global, ORC_T3=global
  wires:
  PS-Simulink Converter15/1 -> To Workspace2/1, Scope15/1
  PS-Simulink Converter5/1 -> To Workspace3/1, Scope7/1, [ORC_P3]
  PS-Simulink Converter1/1 -> To Workspace1/1, Scope1/1
  PS-Simulink Converter2/1 -> To Workspace/1, Scope2/1
  PS-Simulink Converter4/1 -> To Workspace4/1, Scope6/1, [ORC_T3]
  connections:
  PS-Simulink Converter4/LConn1 -- "Pressure, Temperature & Internal Energy Sensor (2P)2"/RConn2
  PS-Simulink Converter15/LConn1 -- Thermodynamic Properties Sensor (2P)2/RConn1
  Thermodynamic Properties Sensor (2P)2/LConn1 -- Conn2/RConn1
  "Pressure, Temperature & Internal Energy Sensor (2P)2"/RConn1 -- PS-Simulink Converter5/LConn1
  "Pressure, Temperature & Internal Energy Sensor (2P)2"/LConn1 -- Conn1/RConn1
  Thermodynamic Properties Sensor (2P)2/RConn3 -- PS-Simulink Converter1/LConn1
  PS-Simulink Converter2/LConn1 -- Thermodynamic Properties Sensor (2P)2/RConn2

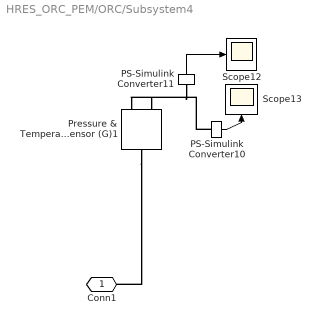
== system HRES_ORC_PEM/ORC/Subsystem4 ==
  PS-Simulink Converter10 : nesl_utility/PS-Simulink Converter  PhysicalDomain=network_engine_domain  SubClassName=ps_output  LeftPortType=input  RightPortType=output  PseudoPeriodic=off  Frequencies=[]  VectorFormat=inherit  Unit=K  AffineConversion=off
  PS-Simulink Converter11 : nesl_utility/PS-Simulink Converter  PhysicalDomain=network_engine_domain  SubClassName=ps_output  LeftPortType=input  RightPortType=output  PseudoPeriodic=off  Frequencies=[]  VectorFormat=inherit  Unit=Pa  AffineConversion=off
  Pressure & Temperature Sensor (G)1 : fl_lib/Gas/Sensors/Pressure & Temperature Sensor (G)  reference=foundation.enum.MeasurementReference.absolute  pressure=true  pressure_spec=foundation.enum.PressureMeasementSpec.Absolute  temperature=true
      settings: InternalSimscapePortConfiguration="{\"Bottom\":[{\"id\":\"T\",\"label\":\"T\",\"type\":\"output\"}],\"Left\":[{\"id\":\"A\",\"label\":\"A\",\"type\":\"foundation.gas.gas\"}],\"Right\":[{\"id\":\"Pa\",\"label\":\"Pa\",\"type\":\"output\"}],\"Top\":[]}"
  Scope12 : Scope
      settings: ActiveDisplayYMinimum=-1  ActiveDisplayYMaximum=1  DataLoggingVariableName=ScopeData12
  Scope13 : Scope
      settings: ActiveDisplayYMinimum=-1  ActiveDisplayYMaximum=1  DataLoggingVariableName=ScopeData13
  Conn1 : PMIOPort  Side=Left
  wires:
  PS-Simulink Converter11/1 -> Scope12/1
  PS-Simulink Converter10/1 -> Scope13/1
  connections:
  PS-Simulink Converter11/LConn1 -- Pressure & Temperature Sensor (G)1/RConn1
  PS-Simulink Converter10/LConn1 -- Pressure & Temperature Sensor (G)1/RConn2
  Pressure & Temperature Sensor (G)1/LConn1 -- Conn1/RConn1

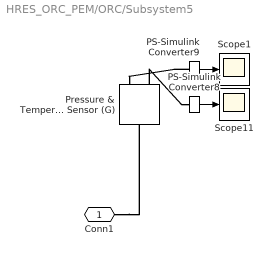
== system HRES_ORC_PEM/ORC/Subsystem5 ==
  PS-Simulink Converter8 : nesl_utility/PS-Simulink Converter  PhysicalDomain=network_engine_domain  SubClassName=ps_output  LeftPortType=input  RightPortType=output  PseudoPeriodic=off  Frequencies=[]  VectorFormat=inherit  Unit=K  AffineConversion=off
  PS-Simulink Converter9 : nesl_utility/PS-Simulink Converter  PhysicalDomain=network_engine_domain  SubClassName=ps_output  LeftPortType=input  RightPortType=output  PseudoPeriodic=off  Frequencies=[]  VectorFormat=inherit  Unit=Pa  AffineConversion=off
  Pressure & Temperature Sensor (G) : fl_lib/Gas/Sensors/Pressure & Temperature Sensor (G)  reference=foundation.enum.MeasurementReference.absolute  pressure=true  pressure_spec=foundation.enum.PressureMeasementSpec.Absolute  temperature=true
      settings: InternalSimscapePortConfiguration="{\"Bottom\":[{\"id\":\"T\",\"label\":\"T\",\"type\":\"output\"}],\"Left\":[{\"id\":\"A\",\"label\":\"A\",\"type\":\"foundation.gas.gas\"}],\"Right\":[{\"id\":\"Pa\",\"label\":\"Pa\",\"type\":\"output\"}],\"Top\":[]}"
  Scope1 : Scope
      settings: ActiveDisplayYMinimum=-1  ActiveDisplayYMaximum=1
  Scope11 : Scope
      settings: ActiveDisplayYMinimum=700.88571594322968  ActiveDisplayYMaximum=716.44585297936726  DataLoggingVariableName=ScopeData11
  Conn1 : PMIOPort  Side=Left
  wires:
  PS-Simulink Converter8/1 -> Scope11/1
  PS-Simulink Converter9/1 -> Scope1/1
  connections:
  Pressure & Temperature Sensor (G)/RConn2 -- PS-Simulink Converter8/LConn1
  PS-Simulink Converter9/LConn1 -- Pressure & Temperature Sensor (G)/RConn1
  Conn1/RConn1 -- Pressure & Temperature Sensor (G)/LConn1
